simulink library "Linkage_Decoupled_Link5"  (R2026a)
settings: Solver=VariableStepAuto
undefined symbols (not defined in the file): Init, Left, Linkage, Visual, X, Y, Z
libraries: sm_lib x56, Suspension_Utilities x23, fl_lib x1, nesl_utility x1
(part 2 of 3)

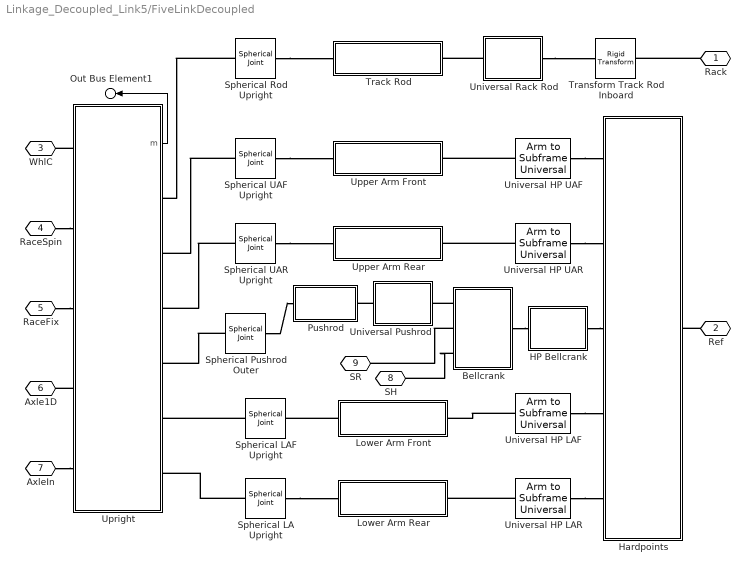
== system Linkage_Decoupled_Link5/FiveLinkDecoupled ==
  Bellcrank : Subsystem  mask(Bellcrank){popup_leftRight=Left, hp_bcr_pivot=hp_bcr_pivot, hp_bcr_shock_heave=hp_bcr_shock_heave, hp_bcr_shock_roll=hp_bcr_shock_roll, hp_pushrod=hp_pushrod_in, bcr_mass=bcr_mass, clr_bcr=clr_bcr, opc_bcr=opc_bcr, radius_bcr=radius_bcr}
      mask prompts: popup_leftRight "Left/Right"; hp_bcr_pivot "HP Bellcrank Pivot [xyz] (m)"; hp_bcr_shock_heave "HP Bellcrank Shock Heave [xyz] (m)"; hp_bcr_shock_roll "HP Bellcrank Shock Roll [xyz] (m)"; hp_pushrod "HP Bellcrank Pushrod [xyz] (m)"; bcr_mass "Mass (kg)"; clr_bcr "Color [RGB]"; opc_bcr "Opacity (0-1)"; radius_bcr "Radius (m)"
      mask help: Models a bellcrank with one pivot and 3 attachment points. The axis of the pivot is normal to the plane formed by the pivot, connection to the pushrod, and connection to the shock.
      mask init:
      | if(popup_leftRight == 1)
      |     rhs_susp = 1;
      |     %hp_shock_roll = hp_bcr_shock_roll; % Use left value
      | elseif(popup_leftRight == 2)
      |     rhs_susp = -1;
      |     % Code to mirror hardpoint about vehicle xz plane 
      |     % and the plane defined by the bellcrank pivot axis
      |     % and the y axis of the vehicle
      |     % Code not used so that points can be specified independently
      |     % Left here as a reference.
      |     %{
      |     a1 = atan2(hp_pushrod(1)-hp_bcr_pivot(1)   ,hp_pushrod(3)-hp_bcr_pivot(3));
      |     a2 = atan2(hp_bcr_shock_roll(1)-hp_bcr_pivot(1),hp_bcr_shock_roll(3)-hp_bcr_pivot(3));
      |     d_roll2piv = norm(hp_bcr_shock_roll([1 3])-hp_bcr_pivot([1 3]));
      |     d_roll_mirror_axis = d_roll2piv*cos(a2-a1);
      |     mirr_dx = d_roll_mirror_axis*sin(a1);
      |     mirr_dz = d_roll_mirror_axis*cos(a1);
      |     hp_shock_roll = ...
      |         [hp_bcr_shock_roll(1)-2*mirr_dx -hp_bcr_shock_roll(2) hp_bcr_shock_roll(3)-2*mirr_dz];
      |     %}
      | end
      | 
      | rhs_hp = [1 rhs_susp 1];
      mask TypeOptions popup_leftRight: Left | Right
      mask TypeOptions clr_bcr: Arm Pivot Shock Roll/clr_solid | Arm Pivot Push/clr_solid | Arm Pivot Shock Heave/clr_solid | Arm Push Shock/clr_solid
      mask TypeOptions opc_bcr: Arm Pivot Shock Roll/opc_solid | Arm Pivot Push/opc_solid | Arm Pivot Shock Heave/opc_solid | Arm Push Shock/opc_solid
      mask TypeOptions radius_bcr: Arm Pivot Shock Roll/rad_solid | Arm Pivot Push/rad_solid | Arm Pivot Shock Heave/rad_solid | Arm Push Shock/rad_solid
      mask DialogControl cont_ua Prompt: UA
      mask DialogControl cont_vis_ua Prompt: Visualization
      mask Display: image('sm_car_vehicle_linkage_bellcrank_IMAGE.png');
  HP Bellcrank : Subsystem  mask(Revolute Joint 3 Points){popup_leftRight=Left, hp_bcr_pivot=hp_bcr_pivot, hp_pushrod_in=hp_pushrod_in, hp_bcr_shock=hp_bcr_shock_heave}
      mask prompts: popup_leftRight "Left/Right"; hp_bcr_pivot "HP Bellcrank Pivot [xyz] (m)"; hp_pushrod_in "HP Pushrod Inner [xyz] (m)"; hp_bcr_shock "HP Bellcrank Shock Heave [xyz] (m)"
      mask help: Revolute Joint with degree of freedom normal to 3 hardpoints.
      mask init:
      | % Set parameter for mirroring (+y or -y)
      | if(popup_leftRight == 1)
      |     rhs_susp = 1;    
      | elseif(popup_leftRight == 2)
      |     rhs_susp = -1;
      | end
      | 
      | rhs_hp = [1 rhs_susp 1];
      mask TypeOptions popup_leftRight: Left | Right
      mask Display: image('sm_car_variant_revolute.png')
  Hardpoints : Subsystem  mask{popup_leftRight=Left, hp_in_f_ua=hp_in_f_ua, hp_in_r_ua=hp_in_r_ua, hp_in_f_la=hp_in_f_la, hp_in_r_la=hp_in_r_la, hp_bellcrank=hp_bcr_pivot, clr_hp=clr_hp, opc_hp=opc_hp, size_hp=size_hp}
      mask prompts: popup_leftRight "Left/Right"; hp_in_f_ua "Upper Arm Front [xyz] (m)"; hp_in_r_ua "Upper Arm Rear [xyz] (m)"; hp_in_f_la "Lower Arm Front [xyz] (m)"; hp_in_r_la "Lower Arm Rear [xyz] (m)"; hp_bellcrank "Bellcrank Pivot [xyz] (m)"
      mask init:
      | % Set parameter for mirroring (+y or -y)
      | if(popup_leftRight == 1)
      |     rhs_susp = 1;    
      | elseif(popup_leftRight == 2)
      |     rhs_susp = -1;
      | end
      | 
      | rhs_hp = [1 rhs_susp 1];
      mask TypeOptions popup_leftRight: Left | Right
      mask TypeOptions clr_hp: Vis HP LAr/GraphicDiffuseColor | Vis HP Bellcrank/GraphicDiffuseColor | Vis HP UAf/GraphicDiffuseColor | Vis HP UAr/GraphicDiffuseColor | Vis HP LAf/GraphicDiffuseColor
      mask TypeOptions opc_hp: Vis HP LAr/GraphicOpacity | Vis HP Bellcrank/GraphicOpacity | Vis HP UAf/GraphicOpacity | Vis HP UAr/GraphicOpacity | Vis HP LAf/GraphicOpacity
      mask DialogControl cont_hp Prompt: Hardpoints
      mask DialogControl cont_vis_hp Prompt: Visualization
      mask DialogControl text_clr_hp Prompt: Color [RGB]
      mask DialogControl text_opc_hp Prompt: Opac. (0-1)
      mask DialogControl text_size_hp Prompt: Size (m)
      mask DialogControl text_hp Prompt: Hardpoints
      mask Display: image('sm_car_vehicle_linkage_link5_hp_IMAGE.png');
  Lower Arm Front : Subsystem  VariantControl=Steer  mask{popup_leftRight=Left, hp_in=hp_in_f_la, hp_out=hp_out_f_la, rod_mass=laf_mass, clr_conn_rod=clr_conn_links, opc_conn_rod=opc_conn_links, size_conn_rod=size_conn_links, clr_rod=clr_laf, opc_rod=opc_laf, radius_rod=radius_laf}
      mask prompts: popup_leftRight "Left/Right"; hp_in "Inboard [xyz] (m)"; hp_out "Outboard [xyz] (m)"; rod_mass "Mass (kg)"
      mask init:
      | if(popup_leftRight == 1)
      |     rhs_rod = 1;
      | elseif(popup_leftRight == 2)
      |     rhs_rod = -1;
      | end
      mask TypeOptions popup_leftRight: Left | Right
      mask TypeOptions rod_mass: Arm/Mass
      mask TypeOptions clr_conn_rod:
      | Vis
      | Upright
      | Steer/GraphicDiffuseColor | Vis
      | Rack
      | Rod/GraphicDiffuseColor
      mask TypeOptions opc_conn_rod:
      | Vis
      | Upright
      | Steer/GraphicOpacity | Vis
      | Rack
      | Rod/GraphicOpacity
      mask TypeOptions clr_rod: Arm/clr_solid
      mask TypeOptions opc_rod: Arm/opc_solid
      mask TypeOptions radius_rod: Arm/rad_solid
      mask DialogControl cont_rod Prompt: Rod
      mask DialogControl grp_rod Prompt: Rod
      mask DialogControl cont_vis_rod Prompt: Visualization
      mask DialogControl text_clr_rod Prompt: Color [RGB]
      mask DialogControl text_opc_rod Prompt: Opacity (0-1)
      mask DialogControl text_size_rod Prompt: Radius (m)
      mask DialogControl text_conn_rod Prompt: Connections
      mask DialogControl text_rod_rod Prompt: Rod
      mask Display: image('sm_car_vehicle_linkage_link_IMAGE.png');
  Lower Arm Rear : Subsystem  VariantControl=Steer  mask{popup_leftRight=Left, hp_in=hp_in_r_la, hp_out=hp_out_r_la, rod_mass=lar_mass, clr_conn_rod=clr_conn_links, opc_conn_rod=opc_conn_links, size_conn_rod=size_conn_links, clr_rod=clr_lar, opc_rod=opc_lar, radius_rod=radius_lar}
      mask prompts: popup_leftRight "Left/Right"; hp_in "Inboard [xyz] (m)"; hp_out "Outboard [xyz] (m)"; rod_mass "Mass (kg)"
      mask init:
      | if(popup_leftRight == 1)
      |     rhs_rod = 1;
      | elseif(popup_leftRight == 2)
      |     rhs_rod = -1;
      | end
      mask TypeOptions popup_leftRight: Left | Right
      mask TypeOptions rod_mass: Arm/Mass
      mask TypeOptions clr_conn_rod:
      | Vis
      | Upright
      | Steer/GraphicDiffuseColor | Vis
      | Rack
      | Rod/GraphicDiffuseColor
      mask TypeOptions opc_conn_rod:
      | Vis
      | Upright
      | Steer/GraphicOpacity | Vis
      | Rack
      | Rod/GraphicOpacity
      mask TypeOptions clr_rod: Arm/clr_solid
      mask TypeOptions opc_rod: Arm/opc_solid
      mask TypeOptions radius_rod: Arm/rad_solid
      mask DialogControl cont_rod Prompt: Rod
      mask DialogControl grp_rod Prompt: Rod
      mask DialogControl cont_vis_rod Prompt: Visualization
      mask DialogControl text_clr_rod Prompt: Color [RGB]
      mask DialogControl text_opc_rod Prompt: Opacity (0-1)
      mask DialogControl text_size_rod Prompt: Radius (m)
      mask DialogControl text_conn_rod Prompt: Connections
      mask DialogControl text_rod_rod Prompt: Rod
      mask Display: image('sm_car_vehicle_linkage_link_IMAGE.png');
  Pushrod : Subsystem  VariantControl=Steer  mask{popup_leftRight=Left, hp_in=hp_pushrod_in, hp_out=hp_pushrod_out, rod_mass=pushrod_mass, clr_conn_rod=clr_conn_pushrod, opc_conn_rod=opc_conn_pushrod, size_conn_rod=size_conn_pushrod, clr_rod=clr_pushrod, opc_rod=opc_pushrod, radius_rod=radius_pushrod}
      mask prompts: popup_leftRight "Left/Right"; hp_in "Inboard [xyz] (m)"; hp_out "Outboard [xyz] (m)"; rod_mass "Mass (kg)"
      mask init:
      | if(popup_leftRight == 1)
      |     rhs_rod = 1;
      | elseif(popup_leftRight == 2)
      |     rhs_rod = -1;
      | end
      mask TypeOptions popup_leftRight: Left | Right
      mask TypeOptions rod_mass: Arm/Mass
      mask TypeOptions clr_conn_rod:
      | Vis
      | Upright
      | Steer/GraphicDiffuseColor | Vis
      | Rack
      | Rod/GraphicDiffuseColor
      mask TypeOptions opc_conn_rod:
      | Vis
      | Upright
      | Steer/GraphicOpacity | Vis
      | Rack
      | Rod/GraphicOpacity
      mask TypeOptions clr_rod: Arm/clr_solid
      mask TypeOptions opc_rod: Arm/opc_solid
      mask TypeOptions radius_rod: Arm/rad_solid
      mask DialogControl cont_rod Prompt: Rod
      mask DialogControl grp_rod Prompt: Rod
      mask DialogControl cont_vis_rod Prompt: Visualization
      mask DialogControl text_clr_rod Prompt: Color [RGB]
      mask DialogControl text_opc_rod Prompt: Opacity (0-1)
      mask DialogControl text_size_rod Prompt: Radius (m)
      mask DialogControl text_conn_rod Prompt: Connections
      mask DialogControl text_rod_rod Prompt: Rod
      mask Display: image('sm_car_vehicle_linkage_link_IMAGE.png');
  Spherical LA Upright : sm_lib/Joints/Spherical Joint  JointMode=Normal  CompositeWrenchDir=FollowerOnBase  CompositeWrenchFrame=BaseFrame  SenseConstraintForce=off  SenseConstraintTorque=off  SenseTotalForce=off  SenseTotalTorque=off  PositionTargetSpecify=off  PositionTargetPriority=High  PositionTargetRotationMethod=None  PositionTargetFollAlignAxisA=+X  PositionTargetBaseAlignAxisA=+Y  PositionTargetFollAlignAxisB=+Y  PositionTargetBaseAlignAxisB=+Z  PositionTargetRotationStandardAxis=+Z  PositionTargetRotationAngle=0.0  PositionTargetRotationAngleUnits=deg  PositionTargetRotationArbitraryAxis=[0 0 1]  PositionTargetRotationSequenceAxes=FollowerAxes  PositionTargetRotationSequence=XYX  PositionTargetRotationSequenceAngles=[0 0 0]  PositionTargetRotationSequenceAnglesUnits=deg  PositionTargetRotationMatrix=[1 0 0; 0 1 0; 0 0 1]  PositionTargetQuaternion=[1 0 0 0]  VelocityTargetSpecify=off  VelocityTargetPriority=High  VelocityTargetValue=[0 0 0]  VelocityTargetValueUnits=deg/s  VelocityTargetInFollowerFrame=on  EqPosRotationMethod=None  EqPosFollAlignAxisA=+X  EqPosBaseAlignAxisA=+Y  EqPosFollAlignAxisB=+Y  EqPosBaseAlignAxisB=+Z  EqPosRotationStandardAxis=+Z  EqPosRotationAngle=0.0  EqPosRotationAngleUnits=deg  EqPosRotationArbitraryAxis=[0 0 1]  EqPosRotationSequenceAxes=FollowerAxes  EqPosRotationSequence=XYX  EqPosRotationSequenceAngles=[0 0 0]  EqPosRotationSequenceAnglesUnits=deg  EqPosRotationMatrix=[1 0 0; 0 1 0; 0 0 1]  EqPosQuaternion=[1 0 0 0]  SpringStiffness=0  SpringStiffnessUnits=N*m/deg  DampingCoefficient=0  DampingCoefficientUnits=N*m/(deg/s)  LowerLimitSpecify=off  LowerLimitBound=15  LowerLimitBoundUnits=deg  LowerLimitStiffness=1e4  LowerLimitStiffnessUnits=N*m/deg  LowerLimitDamping=10  LowerLimitDampingUnits=N*m/(deg/s)  LowerLimitTransitionRegionWidth=0.1  LowerLimitTransitionRegionWidthUnits=deg  UpperLimitSpecify=off  UpperLimitBound=45  UpperLimitBoundUnits=deg  UpperLimitStiffness=1e4  UpperLimitStiffnessUnits=N*m/deg  UpperLimitDamping=10  UpperLimitDampingUnits=N*m/(deg/s)  UpperLimitTransitionRegionWidth=0.1  UpperLimitTransitionRegionWidthUnits=deg  TorqueActuationMode=NoTorque  ActuateTorqueX=off  ActuateTorqueY=off  ActuateTorqueZ=off  ActuateTorque=off  ActuationFrame=BaseFrame  SensePosition=off  SenseVelocityX=off  SenseVelocityY=off  SenseVelocityZ=off  SenseVelocity=off  SenseAccelerationX=off  SenseAccelerationY=off  SenseAccelerationZ=off  SenseAcceleration=off  SenseLowerLimitTorqueMag=off  SenseUpperLimitTorqueMag=off  SensingFrame=BaseFrame
  Spherical LAF Upright : sm_lib/Joints/Spherical Joint  JointMode=Normal  CompositeWrenchDir=FollowerOnBase  CompositeWrenchFrame=BaseFrame  SenseConstraintForce=off  SenseConstraintTorque=off  SenseTotalForce=off  SenseTotalTorque=off  PositionTargetSpecify=off  PositionTargetPriority=High  PositionTargetRotationMethod=None  PositionTargetFollAlignAxisA=+X  PositionTargetBaseAlignAxisA=+Y  PositionTargetFollAlignAxisB=+Y  PositionTargetBaseAlignAxisB=+Z  PositionTargetRotationStandardAxis=+Z  PositionTargetRotationAngle=0.0  PositionTargetRotationAngleUnits=deg  PositionTargetRotationArbitraryAxis=[0 0 1]  PositionTargetRotationSequenceAxes=FollowerAxes  PositionTargetRotationSequence=XYX  PositionTargetRotationSequenceAngles=[0 0 0]  PositionTargetRotationSequenceAnglesUnits=deg  PositionTargetRotationMatrix=[1 0 0; 0 1 0; 0 0 1]  PositionTargetQuaternion=[1 0 0 0]  VelocityTargetSpecify=off  VelocityTargetPriority=High  VelocityTargetValue=[0 0 0]  VelocityTargetValueUnits=deg/s  VelocityTargetInFollowerFrame=on  EqPosRotationMethod=None  EqPosFollAlignAxisA=+X  EqPosBaseAlignAxisA=+Y  EqPosFollAlignAxisB=+Y  EqPosBaseAlignAxisB=+Z  EqPosRotationStandardAxis=+Z  EqPosRotationAngle=0.0  EqPosRotationAngleUnits=deg  EqPosRotationArbitraryAxis=[0 0 1]  EqPosRotationSequenceAxes=FollowerAxes  EqPosRotationSequence=XYX  EqPosRotationSequenceAngles=[0 0 0]  EqPosRotationSequenceAnglesUnits=deg  EqPosRotationMatrix=[1 0 0; 0 1 0; 0 0 1]  EqPosQuaternion=[1 0 0 0]  SpringStiffness=0  SpringStiffnessUnits=N*m/deg  DampingCoefficient=0  DampingCoefficientUnits=N*m/(deg/s)  LowerLimitSpecify=off  LowerLimitBound=15  LowerLimitBoundUnits=deg  LowerLimitStiffness=1e4  LowerLimitStiffnessUnits=N*m/deg  LowerLimitDamping=10  LowerLimitDampingUnits=N*m/(deg/s)  LowerLimitTransitionRegionWidth=0.1  LowerLimitTransitionRegionWidthUnits=deg  UpperLimitSpecify=off  UpperLimitBound=45  UpperLimitBoundUnits=deg  UpperLimitStiffness=1e4  UpperLimitStiffnessUnits=N*m/deg  UpperLimitDamping=10  UpperLimitDampingUnits=N*m/(deg/s)  UpperLimitTransitionRegionWidth=0.1  UpperLimitTransitionRegionWidthUnits=deg  TorqueActuationMode=NoTorque  ActuateTorqueX=off  ActuateTorqueY=off  ActuateTorqueZ=off  ActuateTorque=off  ActuationFrame=BaseFrame  SensePosition=off  SenseVelocityX=off  SenseVelocityY=off  SenseVelocityZ=off  SenseVelocity=off  SenseAccelerationX=off  SenseAccelerationY=off  SenseAccelerationZ=off  SenseAcceleration=off  SenseLowerLimitTorqueMag=off  SenseUpperLimitTorqueMag=off  SensingFrame=BaseFrame
  Spherical Pushrod Outer : sm_lib/Joints/Spherical Joint  JointMode=Normal  CompositeWrenchDir=FollowerOnBase  CompositeWrenchFrame=BaseFrame  SenseConstraintForce=off  SenseConstraintTorque=off  SenseTotalForce=off  SenseTotalTorque=off  PositionTargetSpecify=on  PositionTargetPriority=Low  PositionTargetRotationMethod=AlignedAxes  PositionTargetFollAlignAxisA=+X  PositionTargetBaseAlignAxisA=+X  PositionTargetFollAlignAxisB=+Y  PositionTargetBaseAlignAxisB=+Y  PositionTargetRotationStandardAxis=+Z  PositionTargetRotationAngle=0.0  PositionTargetRotationAngleUnits=deg  PositionTargetRotationArbitraryAxis=[0 0 1]  PositionTargetRotationSequenceAxes=FollowerAxes  PositionTargetRotationSequence=XYX  PositionTargetRotationSequenceAngles=[0 0 0]  PositionTargetRotationSequenceAnglesUnits=deg  PositionTargetRotationMatrix=[1 0 0; 0 1 0; 0 0 1]  PositionTargetQuaternion=[1 0 0 0]  VelocityTargetSpecify=off  VelocityTargetPriority=High  VelocityTargetValue=[0 0 0]  VelocityTargetValueUnits=deg/s  VelocityTargetInFollowerFrame=on  EqPosRotationMethod=None  EqPosFollAlignAxisA=+X  EqPosBaseAlignAxisA=+Y  EqPosFollAlignAxisB=+Y  EqPosBaseAlignAxisB=+Z  EqPosRotationStandardAxis=+Z  EqPosRotationAngle=0.0  EqPosRotationAngleUnits=deg  EqPosRotationArbitraryAxis=[0 0 1]  EqPosRotationSequenceAxes=FollowerAxes  EqPosRotationSequence=XYX  EqPosRotationSequenceAngles=[0 0 0]  EqPosRotationSequenceAnglesUnits=deg  EqPosRotationMatrix=[1 0 0; 0 1 0; 0 0 1]  EqPosQuaternion=[1 0 0 0]  SpringStiffness=0  SpringStiffnessUnits=N*m/deg  DampingCoefficient=0  DampingCoefficientUnits=N*m/(deg/s)  LowerLimitSpecify=off  LowerLimitBound=15  LowerLimitBoundUnits=deg  LowerLimitStiffness=1e4  LowerLimitStiffnessUnits=N*m/deg  LowerLimitDamping=10  LowerLimitDampingUnits=N*m/(deg/s)  LowerLimitTransitionRegionWidth=0.1  LowerLimitTransitionRegionWidthUnits=deg  UpperLimitSpecify=off  UpperLimitBound=45  UpperLimitBoundUnits=deg  UpperLimitStiffness=1e4  UpperLimitStiffnessUnits=N*m/deg  UpperLimitDamping=10  UpperLimitDampingUnits=N*m/(deg/s)  UpperLimitTransitionRegionWidth=0.1  UpperLimitTransitionRegionWidthUnits=deg  TorqueActuationMode=NoTorque  ActuateTorqueX=off  ActuateTorqueY=off  ActuateTorqueZ=off  ActuateTorque=off  ActuationFrame=BaseFrame  SensePosition=off  SenseVelocityX=off  SenseVelocityY=off  SenseVelocityZ=off  SenseVelocity=off  SenseAccelerationX=off  SenseAccelerationY=off  SenseAccelerationZ=off  SenseAcceleration=off  SenseLowerLimitTorqueMag=off  SenseUpperLimitTorqueMag=off  SensingFrame=BaseFrame
  Spherical Rod Upright : sm_lib/Joints/Spherical Joint  JointMode=Normal  CompositeWrenchDir=FollowerOnBase  CompositeWrenchFrame=BaseFrame  SenseConstraintForce=off  SenseConstraintTorque=off  SenseTotalForce=off  SenseTotalTorque=off  PositionTargetSpecify=off  PositionTargetPriority=High  PositionTargetRotationMethod=None  PositionTargetFollAlignAxisA=+X  PositionTargetBaseAlignAxisA=+Y  PositionTargetFollAlignAxisB=+Y  PositionTargetBaseAlignAxisB=+Z  PositionTargetRotationStandardAxis=+Z  PositionTargetRotationAngle=0.0  PositionTargetRotationAngleUnits=deg  PositionTargetRotationArbitraryAxis=[0 0 1]  PositionTargetRotationSequenceAxes=FollowerAxes  PositionTargetRotationSequence=XYX  PositionTargetRotationSequenceAngles=[0 0 0]  PositionTargetRotationSequenceAnglesUnits=deg  PositionTargetRotationMatrix=[1 0 0; 0 1 0; 0 0 1]  PositionTargetQuaternion=[1 0 0 0]  VelocityTargetSpecify=off  VelocityTargetPriority=High  VelocityTargetValue=[0 0 0]  VelocityTargetValueUnits=deg/s  VelocityTargetInFollowerFrame=on  EqPosRotationMethod=None  EqPosFollAlignAxisA=+X  EqPosBaseAlignAxisA=+Y  EqPosFollAlignAxisB=+Y  EqPosBaseAlignAxisB=+Z  EqPosRotationStandardAxis=+Z  EqPosRotationAngle=0.0  EqPosRotationAngleUnits=deg  EqPosRotationArbitraryAxis=[0 0 1]  EqPosRotationSequenceAxes=FollowerAxes  EqPosRotationSequence=XYX  EqPosRotationSequenceAngles=[0 0 0]  EqPosRotationSequenceAnglesUnits=deg  EqPosRotationMatrix=[1 0 0; 0 1 0; 0 0 1]  EqPosQuaternion=[1 0 0 0]  SpringStiffness=0  SpringStiffnessUnits=N*m/deg  DampingCoefficient=0  DampingCoefficientUnits=N*m/(deg/s)  LowerLimitSpecify=off  LowerLimitBound=15  LowerLimitBoundUnits=deg  LowerLimitStiffness=1e4  LowerLimitStiffnessUnits=N*m/deg  LowerLimitDamping=10  LowerLimitDampingUnits=N*m/(deg/s)  LowerLimitTransitionRegionWidth=0.1  LowerLimitTransitionRegionWidthUnits=deg  UpperLimitSpecify=off  UpperLimitBound=45  UpperLimitBoundUnits=deg  UpperLimitStiffness=1e4  UpperLimitStiffnessUnits=N*m/deg  UpperLimitDamping=10  UpperLimitDampingUnits=N*m/(deg/s)  UpperLimitTransitionRegionWidth=0.1  UpperLimitTransitionRegionWidthUnits=deg  TorqueActuationMode=NoTorque  ActuateTorqueX=off  ActuateTorqueY=off  ActuateTorqueZ=off  ActuateTorque=off  ActuationFrame=BaseFrame  SensePosition=off  SenseVelocityX=off  SenseVelocityY=off  SenseVelocityZ=off  SenseVelocity=off  SenseAccelerationX=off  SenseAccelerationY=off  SenseAccelerationZ=off  SenseAcceleration=off  SenseLowerLimitTorqueMag=off  SenseUpperLimitTorqueMag=off  SensingFrame=BaseFrame
  Spherical UAF Upright : sm_lib/Joints/Spherical Joint  JointMode=Normal  CompositeWrenchDir=FollowerOnBase  CompositeWrenchFrame=BaseFrame  SenseConstraintForce=off  SenseConstraintTorque=off  SenseTotalForce=off  SenseTotalTorque=off  PositionTargetSpecify=off  PositionTargetPriority=High  PositionTargetRotationMethod=None  PositionTargetFollAlignAxisA=+X  PositionTargetBaseAlignAxisA=+Y  PositionTargetFollAlignAxisB=+Y  PositionTargetBaseAlignAxisB=+Z  PositionTargetRotationStandardAxis=+Z  PositionTargetRotationAngle=0.0  PositionTargetRotationAngleUnits=deg  PositionTargetRotationArbitraryAxis=[0 0 1]  PositionTargetRotationSequenceAxes=FollowerAxes  PositionTargetRotationSequence=XYX  PositionTargetRotationSequenceAngles=[0 0 0]  PositionTargetRotationSequenceAnglesUnits=deg  PositionTargetRotationMatrix=[1 0 0; 0 1 0; 0 0 1]  PositionTargetQuaternion=[1 0 0 0]  VelocityTargetSpecify=off  VelocityTargetPriority=High  VelocityTargetValue=[0 0 0]  VelocityTargetValueUnits=deg/s  VelocityTargetInFollowerFrame=on  EqPosRotationMethod=None  EqPosFollAlignAxisA=+X  EqPosBaseAlignAxisA=+Y  EqPosFollAlignAxisB=+Y  EqPosBaseAlignAxisB=+Z  EqPosRotationStandardAxis=+Z  EqPosRotationAngle=0.0  EqPosRotationAngleUnits=deg  EqPosRotationArbitraryAxis=[0 0 1]  EqPosRotationSequenceAxes=FollowerAxes  EqPosRotationSequence=XYX  EqPosRotationSequenceAngles=[0 0 0]  EqPosRotationSequenceAnglesUnits=deg  EqPosRotationMatrix=[1 0 0; 0 1 0; 0 0 1]  EqPosQuaternion=[1 0 0 0]  SpringStiffness=0  SpringStiffnessUnits=N*m/deg  DampingCoefficient=0  DampingCoefficientUnits=N*m/(deg/s)  LowerLimitSpecify=off  LowerLimitBound=15  LowerLimitBoundUnits=deg  LowerLimitStiffness=1e4  LowerLimitStiffnessUnits=N*m/deg  LowerLimitDamping=10  LowerLimitDampingUnits=N*m/(deg/s)  LowerLimitTransitionRegionWidth=0.1  LowerLimitTransitionRegionWidthUnits=deg  UpperLimitSpecify=off  UpperLimitBound=45  UpperLimitBoundUnits=deg  UpperLimitStiffness=1e4  UpperLimitStiffnessUnits=N*m/deg  UpperLimitDamping=10  UpperLimitDampingUnits=N*m/(deg/s)  UpperLimitTransitionRegionWidth=0.1  UpperLimitTransitionRegionWidthUnits=deg  TorqueActuationMode=NoTorque  ActuateTorqueX=off  ActuateTorqueY=off  ActuateTorqueZ=off  ActuateTorque=off  ActuationFrame=BaseFrame  SensePosition=off  SenseVelocityX=off  SenseVelocityY=off  SenseVelocityZ=off  SenseVelocity=off  SenseAccelerationX=off  SenseAccelerationY=off  SenseAccelerationZ=off  SenseAcceleration=off  SenseLowerLimitTorqueMag=off  SenseUpperLimitTorqueMag=off  SensingFrame=BaseFrame
  Spherical UAR Upright : sm_lib/Joints/Spherical Joint  JointMode=Normal  CompositeWrenchDir=FollowerOnBase  CompositeWrenchFrame=BaseFrame  SenseConstraintForce=off  SenseConstraintTorque=off  SenseTotalForce=off  SenseTotalTorque=off  PositionTargetSpecify=on  PositionTargetPriority=Low  PositionTargetRotationMethod=AlignedAxes  PositionTargetFollAlignAxisA=+X  PositionTargetBaseAlignAxisA=+X  PositionTargetFollAlignAxisB=+Y  PositionTargetBaseAlignAxisB=+Y  PositionTargetRotationStandardAxis=+Z  PositionTargetRotationAngle=0.0  PositionTargetRotationAngleUnits=deg  PositionTargetRotationArbitraryAxis=[0 0 1]  PositionTargetRotationSequenceAxes=FollowerAxes  PositionTargetRotationSequence=XYX  PositionTargetRotationSequenceAngles=[0 0 0]  PositionTargetRotationSequenceAnglesUnits=deg  PositionTargetRotationMatrix=[1 0 0; 0 1 0; 0 0 1]  PositionTargetQuaternion=[1 0 0 0]  VelocityTargetSpecify=off  VelocityTargetPriority=High  VelocityTargetValue=[0 0 0]  VelocityTargetValueUnits=deg/s  VelocityTargetInFollowerFrame=on  EqPosRotationMethod=None  EqPosFollAlignAxisA=+X  EqPosBaseAlignAxisA=+Y  EqPosFollAlignAxisB=+Y  EqPosBaseAlignAxisB=+Z  EqPosRotationStandardAxis=+Z  EqPosRotationAngle=0.0  EqPosRotationAngleUnits=deg  EqPosRotationArbitraryAxis=[0 0 1]  EqPosRotationSequenceAxes=FollowerAxes  EqPosRotationSequence=XYX  EqPosRotationSequenceAngles=[0 0 0]  EqPosRotationSequenceAnglesUnits=deg  EqPosRotationMatrix=[1 0 0; 0 1 0; 0 0 1]  EqPosQuaternion=[1 0 0 0]  SpringStiffness=0  SpringStiffnessUnits=N*m/deg  DampingCoefficient=0  DampingCoefficientUnits=N*m/(deg/s)  LowerLimitSpecify=off  LowerLimitBound=15  LowerLimitBoundUnits=deg  LowerLimitStiffness=1e4  LowerLimitStiffnessUnits=N*m/deg  LowerLimitDamping=10  LowerLimitDampingUnits=N*m/(deg/s)  LowerLimitTransitionRegionWidth=0.1  LowerLimitTransitionRegionWidthUnits=deg  UpperLimitSpecify=off  UpperLimitBound=45  UpperLimitBoundUnits=deg  UpperLimitStiffness=1e4  UpperLimitStiffnessUnits=N*m/deg  UpperLimitDamping=10  UpperLimitDampingUnits=N*m/(deg/s)  UpperLimitTransitionRegionWidth=0.1  UpperLimitTransitionRegionWidthUnits=deg  TorqueActuationMode=NoTorque  ActuateTorqueX=off  ActuateTorqueY=off  ActuateTorqueZ=off  ActuateTorque=off  ActuationFrame=BaseFrame  SensePosition=off  SenseVelocityX=off  SenseVelocityY=off  SenseVelocityZ=off  SenseVelocity=off  SenseAccelerationX=off  SenseAccelerationY=off  SenseAccelerationZ=off  SenseAcceleration=off  SenseLowerLimitTorqueMag=off  SenseUpperLimitTorqueMag=off  SensingFrame=BaseFrame
  Track Rod : Subsystem  VariantControl=Steer  mask{popup_leftRight=Left, hp_in=hp_in_rod, hp_out=hp_upr_rod, rod_mass=rod_mass, clr_conn_rod=clr_conn_rod, opc_conn_rod=opc_conn_rod, size_conn_rod=size_conn_rod, clr_rod=clr_rod, opc_rod=opc_rod, radius_rod=radius_rod}
      mask prompts: popup_leftRight "Left/Right"; hp_in "Inboard [xyz] (m)"; hp_out "Outboard [xyz] (m)"; rod_mass "Mass (kg)"
      mask init:
      | if(popup_leftRight == 1)
      |     rhs_rod = 1;
      | elseif(popup_leftRight == 2)
      |     rhs_rod = -1;
      | end
      mask TypeOptions popup_leftRight: Left | Right
      mask TypeOptions rod_mass: Rod/Mass
      mask TypeOptions clr_conn_rod:
      | Vis
      | Upright
      | Steer/GraphicDiffuseColor | Vis
      | Rack
      | Rod/GraphicDiffuseColor
      mask TypeOptions opc_conn_rod:
      | Vis
      | Upright
      | Steer/GraphicOpacity | Vis
      | Rack
      | Rod/GraphicOpacity
      mask TypeOptions clr_rod: Rod/clr_solid
      mask TypeOptions opc_rod: Rod/opc_solid
      mask TypeOptions radius_rod: Rod/rad_solid
      mask DialogControl cont_rod Prompt: Rod
      mask DialogControl grp_rod Prompt: Rod
      mask DialogControl cont_vis_rod Prompt: Visualization
      mask DialogControl text_clr_rod Prompt: Color [RGB]
      mask DialogControl text_opc_rod Prompt: Opacity (0-1)
      mask DialogControl text_size_rod Prompt: Radius (m)
      mask DialogControl text_conn_rod Prompt: Connections
      mask DialogControl text_rod_rod Prompt: Rod
      mask Display: image('sm_car_linkage_trackrod_IMAGE.png');
  Transform Track Rod Inboard : sm_lib/Frames and Transforms/Rigid Transform  RotationMethod=None  FollAlignAxisA=+X  BaseAlignAxisA=+Y  FollAlignAxisB=+Y  BaseAlignAxisB=+Z  RotationStandardAxis=+Z  RotationAngle=0.0  RotationAngleUnits=deg  RotationArbitraryAxis=[0 0 1]  RotationSequenceAxes=FollowerAxes  RotationSequence=XYX  RotationSequenceAngles=[0 0 0]  RotationSequenceAnglesUnits=deg  RotationMatrix=[1 0 0; 0 1 0; 0 0 1]  Quaternion=[1 0 0 0]  TranslationMethod=Cartesian  TranslationCartesianOffset=hp_in_rod.*[1 rhs_susp 1]  TranslationCartesianOffsetUnits=m  TranslationStandardAxis=+Z  TranslationStandardOffset=0  TranslationStandardOffsetUnits=m  TranslationROffset=0  TranslationROffsetUnits=m  TranslationThetaOffset=0  TranslationThetaOffsetUnits=deg  TranslationZOffset=0  TranslationZOffsetUnits=m
  Universal HP LAF : Suspension_Utilities/Arm to Subframe Universal  VariantControl=Variant1  LabelModeActiveChoice=Bushing_AxRad  popup_leftRight=Left  hp_joint=hp_in_f_la  Connection=LowerArmF_to_Subframe  VariantLabel=LowerArmF_to_Subframe.class.Value
      settings: AttributesFormatString=%<ActiveVariant>  SourceProductName=SmCar - Suspension Utilites
  Universal HP LAR : Suspension_Utilities/Arm to Subframe Universal  VariantControl=Variant1  LabelModeActiveChoice=Bushing_AxRad  popup_leftRight=Left  hp_joint=hp_in_r_la  Connection=LowerArmR_to_Subframe  VariantLabel=LowerArmR_to_Subframe.class.Value
      settings: AttributesFormatString=%<ActiveVariant>  SourceProductName=SmCar - Suspension Utilites
  Universal HP UAF : Suspension_Utilities/Arm to Subframe Universal  VariantControl=Variant1  LabelModeActiveChoice=Bushing_AxRad  popup_leftRight=Left  hp_joint=hp_in_f_ua  Connection=UpperArmF_to_Subframe  VariantLabel=UpperArmF_to_Subframe.class.Value
      settings: AttributesFormatString=%<ActiveVariant>  SourceProductName=SmCar - Suspension Utilites
  Universal HP UAR : Suspension_Utilities/Arm to Subframe Universal  VariantControl=Variant1  LabelModeActiveChoice=Bushing_AxRad  popup_leftRight=Left  hp_joint=hp_in_r_ua  Connection=UpperArmR_to_Subframe  VariantLabel=UpperArmR_to_Subframe.class.Value
      settings: AttributesFormatString=%<ActiveVariant>  SourceProductName=SmCar - Suspension Utilites
  Universal Pushrod : Subsystem
      mask Display: image('sm_car_variant_universal.png');
  Universal Rack Rod : Subsystem
      mask Display: image('sm_car_variant_universal.png');
  Upper Arm Front : Subsystem  VariantControl=Steer  mask{popup_leftRight=Left, hp_in=hp_in_f_ua, hp_out=hp_out_f_ua, rod_mass=uaf_mass, clr_conn_rod=clr_conn_links, opc_conn_rod=opc_conn_links, size_conn_rod=size_conn_links, clr_rod=clr_uaf, opc_rod=opc_uaf, radius_rod=radius_uaf}
      mask prompts: popup_leftRight "Left/Right"; hp_in "Inboard [xyz] (m)"; hp_out "Outboard [xyz] (m)"; rod_mass "Mass (kg)"
      mask init:
      | if(popup_leftRight == 1)
      |     rhs_rod = 1;
      | elseif(popup_leftRight == 2)
      |     rhs_rod = -1;
      | end
      mask TypeOptions popup_leftRight: Left | Right
      mask TypeOptions rod_mass: Rod/Mass
      mask TypeOptions clr_conn_rod:
      | Vis
      | Upright
      | Steer/GraphicDiffuseColor | Vis
      | Rack
      | Rod/GraphicDiffuseColor
      mask TypeOptions opc_conn_rod:
      | Vis
      | Upright
      | Steer/GraphicOpacity | Vis
      | Rack
      | Rod/GraphicOpacity
      mask TypeOptions clr_rod: Rod/clr_solid
      mask TypeOptions opc_rod: Rod/opc_solid
      mask TypeOptions radius_rod: Rod/rad_solid
      mask DialogControl cont_rod Prompt: Rod
      mask DialogControl grp_rod Prompt: Rod
      mask DialogControl cont_vis_rod Prompt: Visualization
      mask DialogControl text_clr_rod Prompt: Color [RGB]
      mask DialogControl text_opc_rod Prompt: Opac. (0-1)
      mask DialogControl text_size_rod Prompt: Size (m)
      mask DialogControl text_conn_rod Prompt: Connections
      mask DialogControl text_rod_rod Prompt: Rod
      mask Display: image('sm_car_vehicle_linkage_link_IMAGE.png');
  Upper Arm Rear : Subsystem  VariantControl=Steer  mask{popup_leftRight=Left, hp_in=hp_in_r_ua, hp_out=hp_out_r_ua, rod_mass=uar_mass, clr_conn_rod=clr_conn_links, opc_conn_rod=opc_conn_links, size_conn_rod=size_conn_links, clr_rod=clr_uar, opc_rod=opc_uar, radius_rod=radius_uar}
      mask prompts: popup_leftRight "Left/Right"; hp_in "Inboard [xyz] (m)"; hp_out "Outboard [xyz] (m)"; rod_mass "Mass (kg)"
      mask init:
      | if(popup_leftRight == 1)
      |     rhs_rod = 1;
      | elseif(popup_leftRight == 2)
      |     rhs_rod = -1;
      | end
      mask TypeOptions popup_leftRight: Left | Right
      mask TypeOptions rod_mass: Rod/Mass
      mask TypeOptions clr_conn_rod:
      | Vis
      | Upright
      | Steer/GraphicDiffuseColor | Vis
      | Rack
      | Rod/GraphicDiffuseColor
      mask TypeOptions opc_conn_rod:
      | Vis
      | Upright
      | Steer/GraphicOpacity | Vis
      | Rack
      | Rod/GraphicOpacity
      mask TypeOptions clr_rod: Rod/clr_solid
      mask TypeOptions opc_rod: Rod/opc_solid
      mask TypeOptions radius_rod: Rod/rad_solid
      mask DialogControl cont_rod Prompt: Rod
      mask DialogControl grp_rod Prompt: Rod
      mask DialogControl cont_vis_rod Prompt: Visualization
      mask DialogControl text_clr_rod Prompt: Color [RGB]
      mask DialogControl text_opc_rod Prompt: Opac. (0-1)
      mask DialogControl text_size_rod Prompt: Size (m)
      mask DialogControl text_conn_rod Prompt: Connections
      mask DialogControl text_rod_rod Prompt: Rod
      mask Display: image('sm_car_vehicle_linkage_link_IMAGE.png');
  Upright : Subsystem  mask{popup_leftRight=Left, hp_uaf_out=hp_out_f_ua, hp_uar_out=hp_out_r_ua, hp_laf_out=hp_out_f_la, hp_lar_out=hp_out_r_la, hp_pushrod=hp_pushrod_out, hp_upr_rod=hp_upr_rod, hp_upr_cg=hp_upr_cg, hp_upr_wc=hp_upr_wc, axle_len=axle_len, axle_whlc_to_bearing=axle_whlc_to_bearing, axle_mass=axle_mass, atoe=atoe, acamber=acamber, upr_mass=upr_mass, whl_init_spd_upr=whl_init_spd, clr_conn_upr=clr_conn_upr, opc_conn_upr=opc_conn_upr, size_conn_upr=size_conn_upr, clr_upr=clr_upr, opc_upr=opc_upr, radius_upr=radius_upr, clr_axle=clr_axle, opc_axle=opc_axle, radius_axle=radius_axle}
      mask prompts: popup_leftRight "Left/Right"; hp_uaf_out "Upper Arm Front Outboard [xyz] (m)"; hp_uar_out "Upper Arm Rear Outboard [xyz] (m)"; hp_laf_out "Lower Arm Front Outboard [xyz] (m)"; hp_lar_out "Lower Arm Rear Outboard [xyz] (m)"; hp_pushrod "Pushrod Outboard [xyz] (m)"; hp_upr_rod "Track Rod Outboard [xyz] (m)"; hp_upr_cg "Center of Mass [xyz] (m)"; hp_upr_wc "Wheel Center [xyz] (m)"; axle_len "Axle Length (m)"; axle_whlc_to_bearing "Distance Wheel Ctr to Bearing (m)"; axle_mass "Axle Mass (kg)"; atoe "Toe Angle (deg)"; acamber "Camber Angle (deg)"; upr_mass "Upright Mass (kg)"; whl_init_spd_upr "Initial Wheel Speed (rad/s)"
      mask init:
      | % Set parameter for mirroring (+y or -y)
      | if(popup_leftRight == 1)
      |     rhs_upr = 1;
      | elseif(popup_leftRight == 2)
      |     rhs_upr = -1;
      | end
      | rhs_hp = [1 rhs_upr 1];
      | 
      | % Additional hardpoint at center of upright
      | % Used as attachment points for axle and steering arm
      | hp_upr_ctr = (hp_uaf_out+hp_laf_out)/2;
      mask TypeOptions popup_leftRight: Left | Right
      mask TypeOptions axle_mass: Axle/Mass
      mask TypeOptions upr_mass:
      | Inertia
      | CG/Mass
      mask TypeOptions whl_init_spd_upr: Revolute/whl_init_spd_jnt
      mask TypeOptions clr_conn_upr:
      | Vis Upright LAF/GraphicDiffuseColor | Vis Upright UAF/GraphicDiffuseColor | Vis
      | Wheel
      | Center/GraphicDiffuseColor
      mask TypeOptions opc_conn_upr:
      | Vis Upright LAF/GraphicOpacity | Vis Upright UAF/GraphicOpacity | Vis
      | Wheel
      | Center/GraphicOpacity
      mask TypeOptions clr_upr:
      | Upright/clr_solid | Steering Arm/clr_solid | Lower
      | Rear Arm/clr_solid | Upper
      | Rear Arm/clr_solid | Pushrod Conn/clr_solid
      mask TypeOptions opc_upr:
      | Upright/opc_solid | Steering Arm/opc_solid | Lower
      | Rear Arm/opc_solid | Upper
      | Rear Arm/opc_solid | Pushrod Conn/opc_solid
      mask TypeOptions radius_upr:
      | Upright/rad_solid | Steering Arm/rad_solid | Lower
      | Rear Arm/rad_solid | Upper
      | Rear Arm/rad_solid | Pushrod Conn/rad_solid
      mask TypeOptions clr_axle: Axle/GraphicDiffuseColor
      mask TypeOptions opc_axle: Axle/GraphicOpacity
      mask TypeOptions radius_axle: Axle/CylinderRadius
      mask DialogControl cont_upright Prompt: Upright
      mask DialogControl grp_upright Prompt: Initialization
      mask DialogControl cont_vis_upr Prompt: Visualization
      mask DialogControl text_clr_upr Prompt: Color [RGB]
      mask DialogControl text_opc_upr Prompt: Opac. (0-1)
      mask DialogControl text_size_upr Prompt: Size (m)
      mask DialogControl text_conn_upr Prompt: Connections
      mask DialogControl text_upright Prompt: Upright
      mask DialogControl text_axle Prompt: Axle
      mask Display: image('sm_car_vehicle_linkage_link5_upr_IMAGE.png');
  Rack : PMIOPort  Side=Right
  Ref : PMIOPort  Port=2  Side=Right
  WhlC : PMIOPort  Port=3  Side=Left
  RaceSpin : PMIOPort  Port=4  Side=Left
  RaceFix : PMIOPort  Port=5  Side=Left
  Axle1D : PMIOPort  Port=6  Side=Left
  AxleIn : PMIOPort  Port=7  Side=Left
  SH : PMIOPort  Port=8  Side=Left
  SR : PMIOPort  Port=9  Side=Left
  Out Bus Element1 : Outport  VectorParamsAs1DForOutWhenUnconnected=off  PortName=m  Element=Upright
  wires:
  Upright/1(m) -> Out Bus Element1/1
  connections:
  AxleIn/RConn1 -- Upright/LConn5
  RaceFix/RConn1 -- Upright/LConn3
  RaceSpin/RConn1 -- Upright/LConn2
  Universal Rack Rod/LConn1 -- Track Rod/RConn1
  Spherical Rod Upright/LConn1 -- Track Rod/LConn1
  Spherical UAF Upright/RConn1 -- Upright/RConn2
  Lower Arm Front/LConn1 -- Spherical LAF Upright/LConn1
  Spherical LAF Upright/RConn1 -- Upright/RConn5
  Universal HP LAF/RConn1 -- Lower Arm Front/RConn1
  Upright/LConn4 -- Axle1D/RConn1
  Rack/RConn1 -- Transform Track Rod Inboard/LConn1
  Spherical Rod Upright/RConn1 -- Upright/RConn1
  Universal HP UAF/LConn1 -- Hardpoints/LConn1
  Ref/RConn1 -- Hardpoints/RConn1
  HP Bellcrank/LConn1 -- Hardpoints/LConn3
  Upright/LConn1 -- WhlC/RConn1
  Spherical LA Upright/RConn1 -- Upright/RConn6
  Spherical LA Upright/LConn1 -- Lower Arm Rear/LConn1
  Universal HP LAR/LConn1 -- Hardpoints/LConn5
  Universal HP UAR/RConn1 -- Upper Arm Rear/RConn1
  Spherical UAF Upright/LConn1 -- Upper Arm Front/LConn1
  Spherical UAR Upright/LConn1 -- Upper Arm Rear/LConn1
  Spherical UAR Upright/RConn1 -- Upright/RConn3
  Universal HP UAR/LConn1 -- Hardpoints/LConn2
  Universal HP UAF/RConn1 -- Upper Arm Front/RConn1
  Universal HP LAF/LConn1 -- Hardpoints/LConn4
  Universal HP LAR/RConn1 -- Lower Arm Rear/RConn1
  Universal Rack Rod/RConn1 -- Transform Track Rod Inboard/RConn1
  Spherical Pushrod Outer/LConn1 -- Pushrod/LConn1
  Spherical Pushrod Outer/RConn1 -- Upright/RConn4
  Bellcrank/RConn1 -- HP Bellcrank/RConn1
  Bellcrank/LConn3 -- SH/RConn1
  Bellcrank/LConn1 -- Universal Pushrod/RConn1
  Universal Pushrod/LConn1 -- Pushrod/RConn1
  Bellcrank/LConn2 -- SR/RConn1

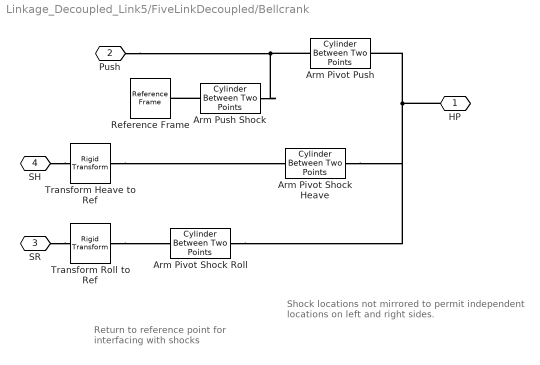
== system Linkage_Decoupled_Link5/FiveLinkDecoupled/Bellcrank ==
  note: Shock locations not mirrored to permit independent locations on left and right sides.
  note: Return to reference point for interfacing with shocks
  Arm Pivot Push : Suspension_Utilities/Cylinder Between Two Points  hp_b=hp_bcr_pivot.*rhs_hp  hp_f=hp_pushrod.*rhs_hp  Mass=bcr_mass/3  clr_solid=clr_bcr  opc_solid=opc_bcr  rad_solid=radius_bcr
      settings: SourceProductName=SmCar - Suspension Utilites
  Arm Pivot Shock Heave : Suspension_Utilities/Cylinder Between Two Points  hp_b=hp_bcr_pivot.*rhs_hp  hp_f=hp_bcr_shock_heave  Mass=bcr_mass/3  clr_solid=clr_bcr  opc_solid=opc_bcr  rad_solid=radius_bcr
      settings: SourceProductName=SmCar - Suspension Utilites
  Arm Pivot Shock Roll : Suspension_Utilities/Cylinder Between Two Points  hp_b=hp_bcr_pivot.*rhs_hp  hp_f=hp_bcr_shock_roll  Mass=bcr_mass*0.001  clr_solid=clr_bcr  opc_solid=opc_bcr  rad_solid=radius_bcr
      settings: SourceProductName=SmCar - Suspension Utilites
  Arm Push Shock : Suspension_Utilities/Cylinder Between Two Points  hp_b=hp_pushrod.*rhs_hp  hp_f=hp_bcr_shock_heave  Mass=bcr_mass/3  clr_solid=clr_bcr  opc_solid=opc_bcr  rad_solid=radius_bcr
      settings: SourceProductName=SmCar - Suspension Utilites
  Reference Frame : sm_lib/Frames and Transforms/Reference Frame
  Transform Heave to Ref : sm_lib/Frames and Transforms/Rigid Transform  RotationMethod=None  FollAlignAxisA=+X  BaseAlignAxisA=+Y  FollAlignAxisB=+Y  BaseAlignAxisB=+Z  RotationStandardAxis=+Z  RotationAngle=0.0  RotationAngleUnits=deg  RotationArbitraryAxis=[0 0 1]  RotationSequenceAxes=FollowerAxes  RotationSequence=XYX  RotationSequenceAngles=[0 0 0]  RotationSequenceAnglesUnits=deg  RotationMatrix=[1 0 0; 0 1 0; 0 0 1]  Quaternion=[1 0 0 0]  TranslationMethod=Cartesian  TranslationCartesianOffset=hp_bcr_shock_heave  TranslationCartesianOffsetUnits=m  TranslationStandardAxis=+Z  TranslationStandardOffset=0  TranslationStandardOffsetUnits=m  TranslationROffset=0  TranslationROffsetUnits=m  TranslationThetaOffset=0  TranslationThetaOffsetUnits=deg  TranslationZOffset=0  TranslationZOffsetUnits=m
  Transform Roll to Ref : sm_lib/Frames and Transforms/Rigid Transform  RotationMethod=None  FollAlignAxisA=+X  BaseAlignAxisA=+Y  FollAlignAxisB=+Y  BaseAlignAxisB=+Z  RotationStandardAxis=+Z  RotationAngle=0.0  RotationAngleUnits=deg  RotationArbitraryAxis=[0 0 1]  RotationSequenceAxes=FollowerAxes  RotationSequence=XYX  RotationSequenceAngles=[0 0 0]  RotationSequenceAnglesUnits=deg  RotationMatrix=[1 0 0; 0 1 0; 0 0 1]  Quaternion=[1 0 0 0]  TranslationMethod=Cartesian  TranslationCartesianOffset=hp_bcr_shock_roll  TranslationCartesianOffsetUnits=m  TranslationStandardAxis=+Z  TranslationStandardOffset=0  TranslationStandardOffsetUnits=m  TranslationROffset=0  TranslationROffsetUnits=m  TranslationThetaOffset=0  TranslationThetaOffsetUnits=deg  TranslationZOffset=0  TranslationZOffsetUnits=m
  HP : PMIOPort  Side=Right
  Push : PMIOPort  Port=2  Side=Left
  SR : PMIOPort  Port=3  Side=Left
  SH : PMIOPort  Port=4  Side=Left
  connections:
  Transform Heave to Ref/RConn1 -- Arm Pivot Shock Heave/RConn1
  Transform Roll to Ref/RConn1 -- Arm Pivot Shock Roll/RConn1
  Arm Push Shock/RConn1 -- Reference Frame/RConn1
  SH/RConn1 -- Transform Heave to Ref/LConn1
  HP/RConn1 -- Arm Pivot Push/LConn1 -- Arm Pivot Shock Roll/LConn1 -- Arm Pivot Shock Heave/LConn1
  Push/RConn1 -- Arm Pivot Push/RConn1 -- Arm Push Shock/LConn1
  SR/RConn1 -- Transform Roll to Ref/LConn1

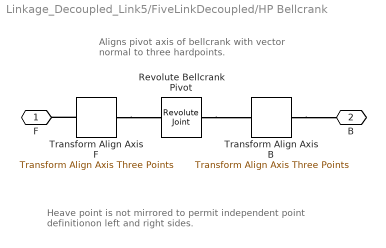
== system Linkage_Decoupled_Link5/FiveLinkDecoupled/HP Bellcrank ==
  note: Heave point is not mirrored to permit independent point definitionon left and right sides.
  note: Aligns pivot axis of bellcrank with vector normal to three hardpoints.
  Revolute Bellcrank Pivot : sm_lib/Joints/Revolute Joint  JointMode=Normal  CompositeWrenchDir=FollowerOnBase  CompositeWrenchFrame=BaseFrame  SenseConstraintForce=off  SenseConstraintTorque=off  SenseTotalForce=off  SenseTotalTorque=off  PositionTargetSpecify=off  PositionTargetPriority=Low  PositionTargetValue=0  PositionTargetValueUnits=deg  VelocityTargetSpecify=off  VelocityTargetPriority=High  VelocityTargetValue=0  VelocityTargetValueUnits=deg/s  EquilibriumPosition=0  EquilibriumPositionUnits=deg  SpringStiffness=0  SpringStiffnessUnits=N*m/deg  DampingCoefficient=0  DampingCoefficientUnits=N*m/(deg/s)  LowerLimitSpecify=off  LowerLimitBound=-90  LowerLimitBoundUnits=deg  LowerLimitStiffness=1e4  LowerLimitStiffnessUnits=N*m/deg  LowerLimitDamping=10  LowerLimitDampingUnits=N*m/(deg/s)  LowerLimitTransitionRegionWidth=0.1  LowerLimitTransitionRegionWidthUnits=deg  UpperLimitSpecify=off  UpperLimitBound=90  UpperLimitBoundUnits=deg  UpperLimitStiffness=1e4  UpperLimitStiffnessUnits=N*m/deg  UpperLimitDamping=10  UpperLimitDampingUnits=N*m/(deg/s)  UpperLimitTransitionRegionWidth=0.1  UpperLimitTransitionRegionWidthUnits=deg  TorqueActuationMode=NoTorque  MotionActuationMode=ComputedMotion  SensePosition=off  SenseVelocity=off  SenseAcceleration=off  SenseTorqueForce=off  SenseLowerLimitTorqueForce=off  SenseUpperLimitTorqueForce=off
  Transform Align Axis B : Suspension_Utilities/Transform Align Axis Three Points  pt1=hp_bcr_pivot.*rhs_hp  pt2=hp_pushrod_in.*rhs_hp  pt3=hp_bcr_shock  popup_f_axis=+Z
      settings: SourceProductName=SmCar - Suspension Utilites
  Transform Align Axis F : Suspension_Utilities/Transform Align Axis Three Points  pt1=hp_bcr_pivot.*rhs_hp  pt2=hp_pushrod_in.*rhs_hp  pt3=hp_bcr_shock  popup_f_axis=+Z
      settings: SourceProductName=SmCar - Suspension Utilites
  F : PMIOPort  Side=Right
  B : PMIOPort  Port=2  Side=Left
  connections:
  Transform Align Axis F/LConn1 -- F/RConn1
  Revolute Bellcrank Pivot/LConn1 -- Transform Align Axis B/RConn1
  Transform Align Axis F/RConn1 -- Revolute Bellcrank Pivot/RConn1
  Transform Align Axis B/LConn1 -- B/RConn1
